simulink model "TEST_ALL"  (R2025b)
settings: Solver=FixedStepAuto  StartTime=0.0  StopTime=inf  RelTol=1e-3  EnableMultiTasking=on
libraries: arduinomotorcarrierlib x4, arduinosensorlib x1, simulink x1, eeGeneralControl x1
settings Model: ExtModeTrigDuration=2  Creator=bkhusain  LastModifiedBy=inggi
settings SolverCC: AlgebraicLoopSolver=TrustRegion
settings OptimizationCC: EnhancedBackFolding=on  PassReuseOutputArgsAs=Individual arguments  ZeroExternalMemoryAtStartup=off  ZeroInternalMemoryAtStartup=off  MaxStackSize=64  OptimizeBlockOrder=speed  DifferentSizesBufferReuse=on  OptimizationCustomize=off  EfficientTunableParamExpr=on
settings DebuggingCC: ParameterTunabilityLossMsg=error  UnconnectedInputMsg=warning  UnconnectedOutputMsg=warning  UnconnectedLineMsg=warning
settings HardwareCC: ProdBitPerPointer=32.0  ProdBitPerSizeT=32.0  ProdBitPerPtrDiffT=32.0  ProdLargestAtomicInteger=Long  ProdLargestAtomicFloat=Double  ProdWordSize=32.0  ProdHWDeviceType=ARM Compatible->ARM Cortex
settings ModelReferenceCC: EnableRefExpFcnMdlSchedulingChecks=on
settings SFSimCC: MATLABDynamicMemAlloc=off
settings RTWCC: SystemTargetFile=ert.tlc  HardwareBoard=Arduino Nano 33 IoT  TemplateMakefile=ert_default_tmf  Toolchain=Arduino ARM  BuildConfiguration=Faster Runs  GPUComputeCapability=3.5  Description=Embedded Coder
settings CodeAppCC: ForceParamTrailComments=on  IgnoreCustomStorageClasses=off  OperatorAnnotations=on  SimulinkDataObjDesc=on  SFDataObjDesc=on  InsertBlockDesc=on
settings ERTTargetCC: ExtModeStaticAllocSize=8192.0  InlinedParameterPlacement=Hierarchical  DynamicArrayContainerType=coder::array  SupportContinuousTime=on  SupportVariableSizeSignals=on

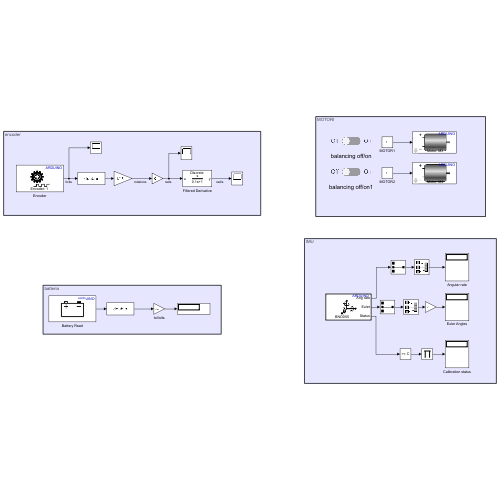
[thumbnail: Simulink's stored preview of the top-level diagram]
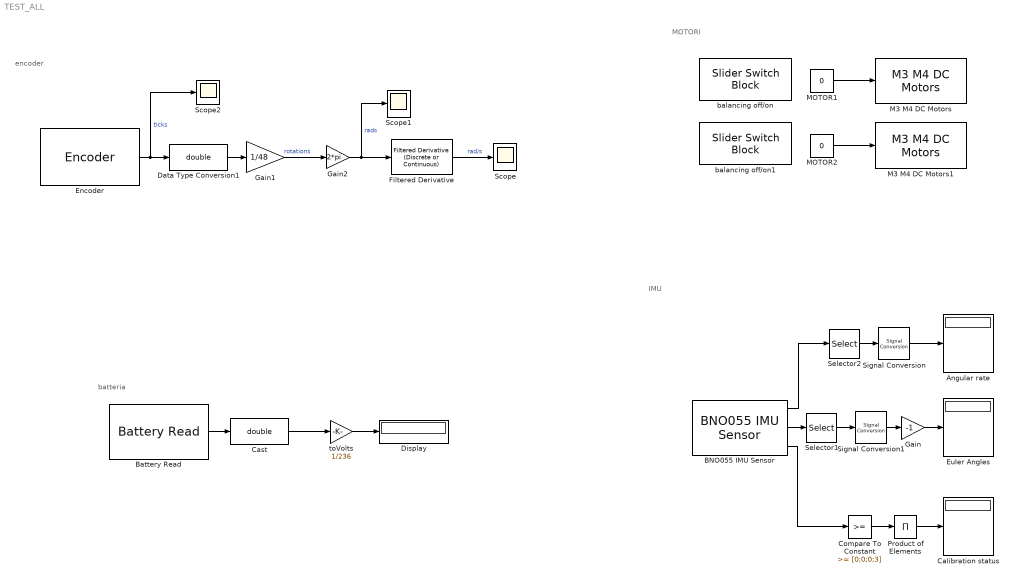
== system TEST_ALL ==
  note: MOTORI
  note: batteria
  note: encoder
  note: IMU
  Angular rate : Display
  BNO055 IMU Sensor : arduinosensorlib/BNO055 IMU Sensor  I2CModule=0  SlaveAddress=0x28  OperationMode=Fusion  Accel=off  AngularRate=on  MagField=off  EulerAngles=on  Quat=off  LinearAccel=off  GravityVector=off  Status=on  Timestamp=off  AccelRange=4G  AccelBW=62.5 Hz  GyroRange=2000 dps  GyroBW=32 Hz  MagODR=10 Hz  spf=1  SampleTime=0.01  blockPlatform=ARDUINO  QueueSizeFactor=1
  Battery Read : arduinomotorcarrierlib/Battery Read  SlaveAddress=uint8( hex2dec( '66' ) )  blockPlatform=ARDUINO  SampleTime=0.01
  Calibration status : Display
  Cast : DataTypeConversion  OutDataTypeStr=double  SaturateOnIntegerOverflow=off  RndMeth=Floor
  Compare To Constant : simulink/Logic and Bit Operations/Compare To Constant  relop=>=  const=[0;0;0;3]  OutDataTypeStr=boolean
  Data Type Conversion1 : DataTypeConversion  OutDataTypeStr=double  SaturateOnIntegerOverflow=off  RndMeth=Floor
  Display : Display
  Encoder : arduinomotorcarrierlib/Encoder  SlaveAddress=uint8( hex2dec( '66' ) )  blockPlatform=ARDUINO  Encoder=1  ShowSpeed=off  ResetOption=on  SampleTime=0.01
  Euler Angles : Display
  "Filtered Derivative " : eeGeneralControl/Filtered Derivative (Discrete or Continuous)  K=1  T=0.1  B=inf  A=-inf  minRatio=10  init_option=Inherited from block input  x0=0  Ts=0.01
  Gain : Gain  Gain=-1
  Gain1 : Gain  Gain=1/48
  Gain2 : Gain  Gain=2*pi
  M3 M4 DC Motors : arduinomotorcarrierlib/M3 M4 DC Motors  MotorNumber=M3  forwardPinNumber=3  reversePinNumber=2
  M3 M4 DC Motors1 : arduinomotorcarrierlib/M3 M4 DC Motors  MotorNumber=M4  forwardPinNumber=4  reversePinNumber=5
  MOTOR1 : Constant  Value=0
  MOTOR2 : Constant  Value=0
  Product of Elements : Product  Inputs=*
  Scope : Scope
      settings: ActiveDisplayYMinimum=-3.7243737075501823E+9  ActiveDisplayYMaximum=3.4263721922272034E+9
  Scope1 : Scope
      settings: ActiveDisplayYMinimum=-3.7243737075501823E+9  ActiveDisplayYMaximum=3.4263721922272034E+9
  Scope2 : Scope
      settings: DataLoggingVariableName=ScopeData2
  Selector1 : Selector  InputPortWidth=3  IndexOptions=Index vector (dialog)  Indices=[2]  OutputSizes=1
  Selector2 : Selector  InputPortWidth=3  IndexOptions=Index vector (dialog)  Indices=[2]  OutputSizes=1
  Signal Conversion : SignalConversion  OverrideOpt=off
  Signal Conversion1 : SignalConversion  OverrideOpt=off
  balancing off/on : SliderSwitchBlock  LabelPosition=Hide
  balancing off/on1 : SliderSwitchBlock  LabelPosition=Hide
  toVolts : Gain  Gain=1/236
  wires:
  MOTOR1/1 -> M3 M4 DC Motors/1
  MOTOR2/1 -> M3 M4 DC Motors1/1
  Battery Read/1 -> Cast/1
  toVolts/1 -> Display/1
  Cast/1 -> toVolts/1
  Gain2/1 -> "Filtered Derivative "/1, Scope1/1  "rads"
  Encoder/1 -> Scope2/1, Data Type Conversion1/1  "ticks"
  "Filtered Derivative "/1 -> Scope/1  "rad/s"
  Gain1/1 -> Gain2/1  "rotations"
  Data Type Conversion1/1 -> Gain1/1
  BNO055 IMU Sensor/2 -> Selector1/1
  Signal Conversion1/1 -> Gain/1
  BNO055 IMU Sensor/3 -> Compare To Constant/1
  Gain/1 -> Euler Angles/1
  Selector2/1 -> Signal Conversion/1
  Product of Elements/1 -> Calibration status/1
  Selector1/1 -> Signal Conversion1/1
  Compare To Constant/1 -> Product of Elements/1
  BNO055 IMU Sensor/1 -> Selector2/1
  Signal Conversion/1 -> Angular rate/1
